simulink model "course_lab2_pd"  (R2024b)
settings: Solver=ode45  StartTime=0.0  StopTime=5  MaxStep=0.003333333333333334  RelTol=1e-7  AbsTol=1e-9
model workspace (MAT data in the model file):
  A = 1
  K = 1
  T = 0.1
  Tf = 0.01
  den = [0.01 1]
  frequency = 1
  num = [0.11 1]
  web_input = timeseries
  web_input.Name = 'unnamed'
  web_input.DataInfo = tsdata.datametadata
  web_input.DataInfo.Interpolation = tsdata.interpolation
  web_input.DataInfo.Interpolation.Fhandle : function handle (value not decoded)
  web_input.DataInfo.Interpolation.Name = 'linear'
  web_input.TimeInfo = tsdata.timemetadata
  web_input.TimeInfo.Length = 1501
  web_input.TimeInfo.DuplicateTimes = 0
  web_input.TimeInfo.Time_ = [0 0.00333333333333 0.00666666666667 0.01 0.0133333333333 0.0166666666667 0.02 0.0233333333333 0.0266666666667 0.03 0.0333333333333 0.0366666666667 ... (1501 elements, 1501x1)]
  web_input.TimeInfo.Initialized = 1
  web_input.QualityInfo = tsdata.qualmetadata
  web_input.Data_ = [1 1 1 1 1 1 1 1 1 1 1 1 ... (1501 elements, 1501x1)]
settings Model: Creator=33657  LastModifiedBy=33657

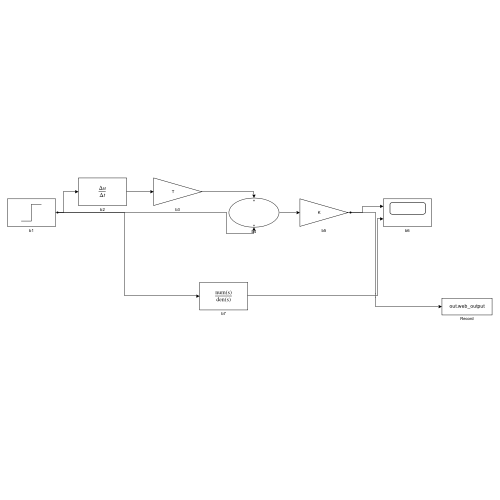
[thumbnail: Simulink's stored preview of the top-level diagram]
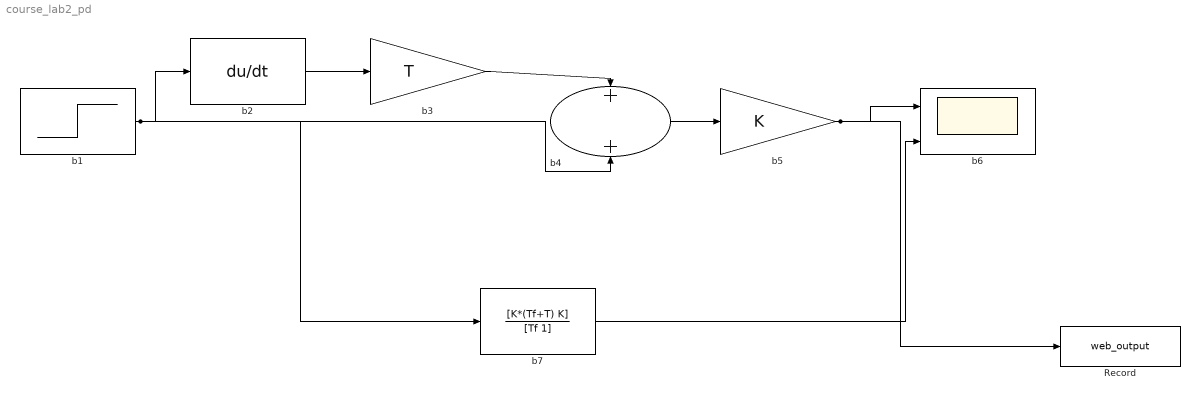
== system course_lab2_pd ==
  Record : ToWorkspace  VariableName=web_output  SaveFormat=Timeseries  SampleTime=-1
  b1 : Step  Time=0  After=A  SampleTime=0
  b2 : Derivative
  b3 : Gain  Gain=T
  b4 : Sum
  b5 : Gain  Gain=K
  b6 : Scope  NumInputPorts=2
  b7 : TransferFcn  Numerator=[K*(Tf+T) K]  Denominator=[Tf 1]
  wires:
  b1/1 -> b2/1, b4/2, b7/1
  b2/1 -> b3/1
  b3/1 -> b4/1
  b4/1 -> b5/1
  b5/1 -> b6/1, Record/1
  b7/1 -> b6/2
